simulink model "ssc_hydromech_power_split_cvt_engine_signal_intf"  (R2025a)
settings: Solver=ode23t  StartTime=0.0  StopTime=70  RelTol=1e-3  AbsTol=1e-3
StartFcn:
  | tic
StopFcn:
  | Elapsed_Sim_Time = toc;
  | disp(['Elapsed Sim Time = ' num2str(Elapsed_Sim_Time)]);
undefined symbols (not defined in the file): DiscIntNeverNeededParam, HMPST, K, Lambda, tau, x0
libraries: fl_lib x30, nesl_utility x16, sm_wheel_loader_lib x9, simulink x7, simulink_extras x6, sdl_lib x3
(part 4 of 4)

== stateflow chart ssc_hydromech_power_split_cvt_engine_signal_intf/CVT/Other/CVT Ratio Ctrl/Clutch Truth Table ==
  state ClutchLogic
    during:
    [K1Actv,K2Actv,K3Actv,K4Actv,KbActv] = ClutchTable(Range);
    state Rest
      during:
      KvActv = 0;
      KrActv = 0;
    state Fwd
      during:
      KvActv = 1;
      KrActv = 0;
    state Rev
      during:
      KvActv = 0;
      KrActv = 1;
    (default) -> (junction 53)
    (junction 53) -> Rev [order 2] : [CmdVehSpdDir==-1]
    (junction 53) -> Fwd [order 3]
    (junction 53) -> Rest [order 1] : [CmdVehSpdDir==0]
    Fwd -> Rest : [CmdVehSpdDir~=1]
    Rev -> Rest : [CmdVehSpdDir~=-1]
    Rest -> Fwd [order 1] : [CmdVehSpdDir==1]
    Rest -> Rev [order 2] : [CmdVehSpdDir==-1]
  data: R function_input; K1 function_output; K2 function_output; K3 function_output; K4 function_output; Kb function_output; Range input; K1Actv output; K2Actv output; K3Actv output; K4Actv output; KbActv output; KvActv output; KrActv output; CmdVehSpdDir input
  function [K1,K2,K3,K4,Kb] = ClutchTable(R):
    | function [K1,K2,K3,K4,Kb] = ClutchTable(R)
    | 
    | aVarTruthTableCondition_1 = false;
    | aVarTruthTableCondition_2 = false;
    | aVarTruthTableCondition_3 = false;
    | aVarTruthTableCondition_4 = false;
    | 
    | 
    | % Range1
    | 
    | aVarTruthTableCondition_1 = logical(R == 1);
    | 
    | % Range2
    | 
    | aVarTruthTableCondition_2 = logical(R == 2);
    | 
    | % Range3
    | 
    | aVarTruthTableCondition_3 = logical(R == 3);
    | 
    | % Range4
    | 
    | aVarTruthTableCondition_4 = logical(R == 4);
    | 
    | if (aVarTruthTableCondition_1 && ~aVarTruthTableCondition_2 && ~aVarTruthTableCondition_3 && ~aVarTruthTableCondition_4)
    |     A1();
    | elseif (~aVarTruthTableCondition_1 && aVarTruthTableCondition_2 && ~aVarTruthTableCondition_3 && ~aVarTruthTableCondition_4)
    |     A2();
    | elseif (~aVarTruthTableCondition_1 && ~aVarTruthTableCondition_2 && aVarTruthTableCondition_3 && ~aVarTruthTableCondition_4)
    |     A3();
    | elseif (~aVarTruthTableCondition_1 && ~aVarTruthTableCondition_2 && ~aVarTruthTableCondition_3 && aVarTruthTableCondition_4)
    |     A4();
    | else % Default
    |     A5();
    | end
    | 
    | function A1()
    | 
    | % ClutchCtrlR1
    | 
    | K1 = 1; K2 = 0; K3 = 0; K4 = 0; Kb = 1;
    | 
    | function A2()
    | 
    | % ClutchCtrlR2
    | 
    | K1 = 0; K2 = 1; K3 = 0; K4 = 0; Kb = 1;
    | 
    | function A3()
    | 
    | % ClutchCtrlR3
    | 
    | K1 = 0; K2 = 1; K3 = 1; K4 = 0; Kb = 0;
    | 
    | function A4()
    | 
    | % ClutchCtrlR4
    | 
    | K1 = 0; K2 = 1; K3 = 0; K4 = 1; Kb = 0;
    | 
    | function A5()
    | 
    | % Default
    | 
    | K1 = 0; K2 = 0; K3 = 0; K4 = 0; Kb = 0;
